simulink model "DIGITAL_WATCH"  (R2026b)
settings: Solver=VariableStepAuto  StopTime=16
libraries: simulink_extras x4
settings Model: Creator=Trealer  LastModifiedBy=Trealer

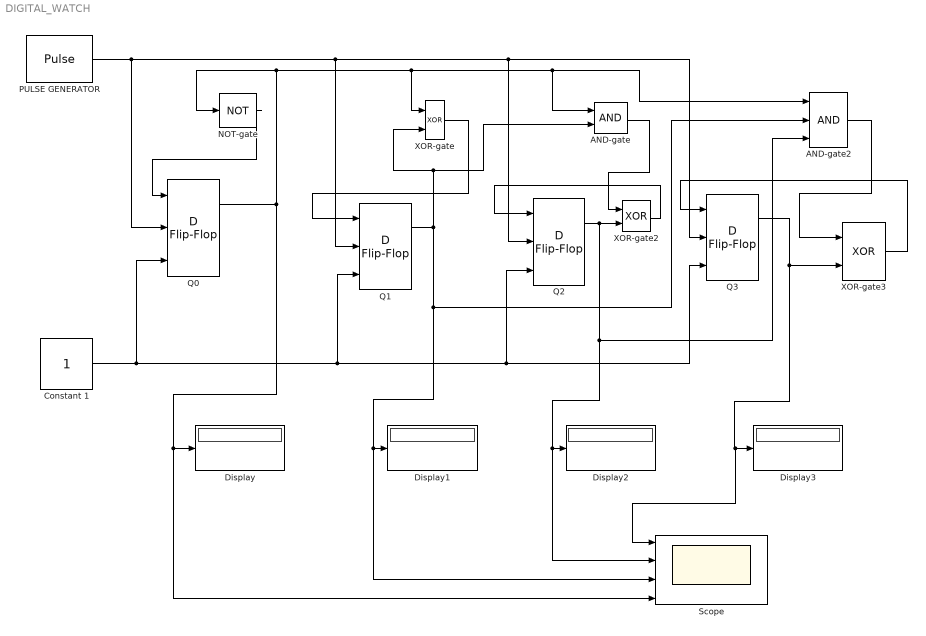
== system DIGITAL_WATCH ==
  AND-gate : Logic  IconShape=distinctive  AllPortsSameDT=off  OutDataTypeStr=boolean
  AND-gate2 : Logic  Inputs=3  IconShape=distinctive  AllPortsSameDT=off  OutDataTypeStr=boolean
  Constant 1 : Constant
  Display{,1..3} (4 alike) : Display
  NOT-gate : Logic  Operator=NOT  IconShape=distinctive  AllPortsSameDT=off  OutDataTypeStr=boolean
  PULSE GENERATOR : DiscretePulseGenerator  PulseType=Time based  Period=1  PulseWidth=50
  Q{0..3} (4 alike) : simulink_extras/Flip Flops/D Flip-Flop
  Scope : Scope  NumInputPorts=4
      settings: ActiveDisplayYMinimum=-0.12499999999999997  ActiveDisplayYMaximum=1.125
  XOR-gate : Logic  Operator=XOR  IconShape=distinctive  AllPortsSameDT=off  OutDataTypeStr=boolean
  XOR-gate2 : Logic  Operator=XOR  IconShape=distinctive  AllPortsSameDT=off  OutDataTypeStr=boolean
  XOR-gate3 : Logic  Operator=XOR  IconShape=distinctive  AllPortsSameDT=off  OutDataTypeStr=boolean
  wires:
  PULSE GENERATOR/1 -> Q1/2, Q3/2, Q2/2, Q0/2
  Constant 1/1 -> Q3/3, Q2/3, Q1/3, Q0/3
  Q0/1 -> Scope/4, Display/1, AND-gate2/1, AND-gate/1, XOR-gate/1, NOT-gate/1
  NOT-gate/1 -> Q0/1
  Q1/1 -> AND-gate/2, XOR-gate/2, Scope/3, Display1/1, AND-gate2/2
  XOR-gate/1 -> Q1/1
  AND-gate/1 -> XOR-gate2/1
  Q2/1 -> Scope/2, Display2/1, AND-gate2/3, XOR-gate2/2
  XOR-gate2/1 -> Q2/1
  AND-gate2/1 -> XOR-gate3/1
  Q3/1 -> Scope/1, Display3/1, XOR-gate3/2
  XOR-gate3/1 -> Q3/1
